simulink model "hrg_wa_v9_bias_reference"  (R2025a)
settings: Solver=ode4  StartTime=0.0  StopTime=0.2  FixedStep=6.2500000000000005e-07  RelTol=1e-3
settings Model: Creator=11725  LastModifiedBy=11725

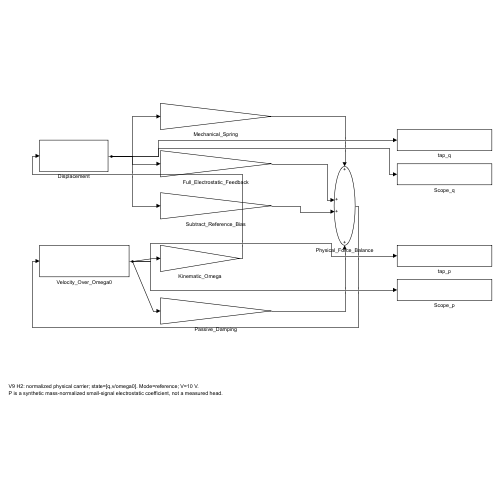
[thumbnail: Simulink's stored preview of the top-level diagram]
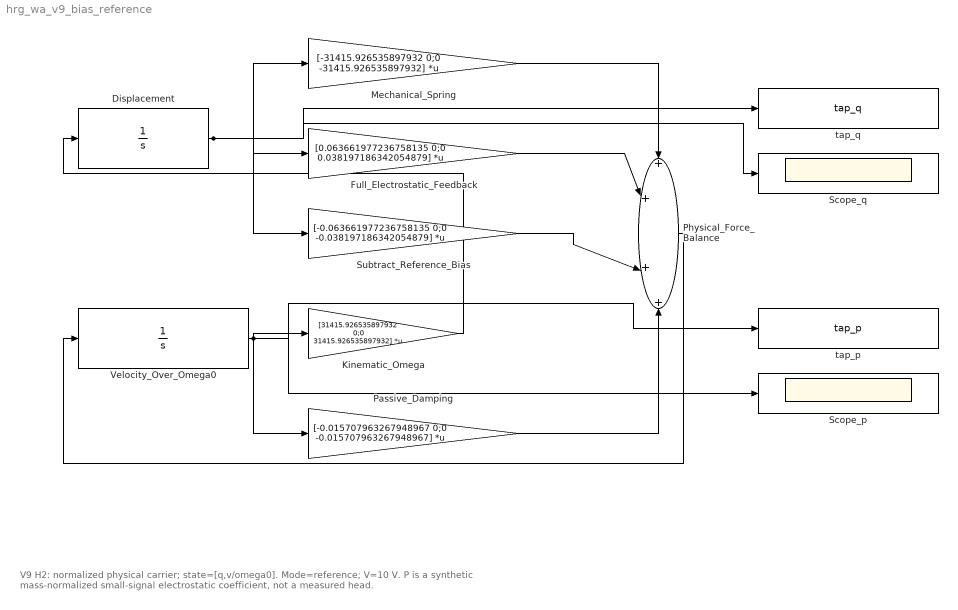
== system hrg_wa_v9_bias_reference ==
  note: V9 H2: normalized physical carrier; state=[q,v/omega0]. Mode=reference; V=10 V.
      | P is a synthetic mass-normalized small-signal electrostatic coefficient, not a measured head.
  Displacement : Integrator  InitialCondition=[0.8;0.6]
  Full_Electrostatic_Feedback : Gain  Gain=[0.063661977236758135 0;0 0.038197186342054879]  Multiplication=Matrix(K*u)
  Kinematic_Omega : Gain  Gain=[31415.926535897932 0;0 31415.926535897932]  Multiplication=Matrix(K*u)
  Mechanical_Spring : Gain  Gain=[-31415.926535897932 0;0 -31415.926535897932]  Multiplication=Matrix(K*u)
  Passive_Damping : Gain  Gain=[-0.015707963267948967 0;0 -0.015707963267948967]  Multiplication=Matrix(K*u)
  Physical_Force_Balance : Sum  Inputs=++++
  Scope_p : Scope
  Scope_q : Scope
  Subtract_Reference_Bias : Gain  Gain=[-0.063661977236758135 0;0 -0.038197186342054879]  Multiplication=Matrix(K*u)
  Velocity_Over_Omega0 : Integrator  InitialCondition=[0;0]
  tap_p : ToWorkspace  VariableName=tap_p  SaveFormat=Timeseries  SampleTime=-1
  tap_q : ToWorkspace  VariableName=tap_q  SaveFormat=Timeseries  SampleTime=-1
  wires:
  Velocity_Over_Omega0/1 -> Kinematic_Omega/1, Passive_Damping/1, tap_p/1, Scope_p/1
  Kinematic_Omega/1 -> Displacement/1
  Displacement/1 -> Mechanical_Spring/1, Full_Electrostatic_Feedback/1, Subtract_Reference_Bias/1, tap_q/1, Scope_q/1
  Mechanical_Spring/1 -> Physical_Force_Balance/1
  Full_Electrostatic_Feedback/1 -> Physical_Force_Balance/2
  Subtract_Reference_Bias/1 -> Physical_Force_Balance/3
  Passive_Damping/1 -> Physical_Force_Balance/4
  Physical_Force_Balance/1 -> Velocity_Over_Omega0/1
